simulink model "OFDM_USRP_Tx_Start"  (R2026a)
settings: Solver=FixedStepDiscrete  StopTime=inf  EnableMultiTasking=on
model workspace: external: MAT-File (data not in the file)
libraries: commdigbbndpm3 x2, dspxfrm3 x1, commfilt2 x1
settings Model: SimulationMode=accelerator  Creator=thua3267  LastModifiedBy=dawn

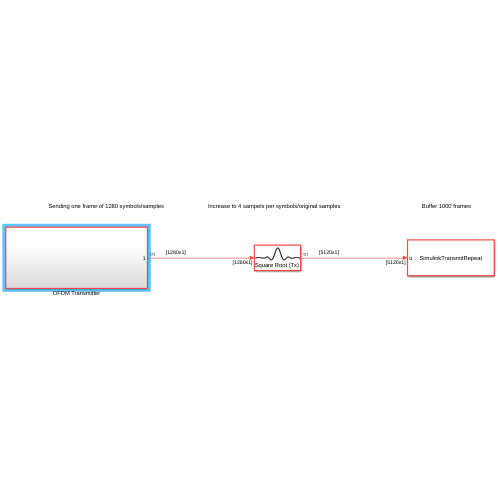
[thumbnail: Simulink's stored preview of the top-level diagram]
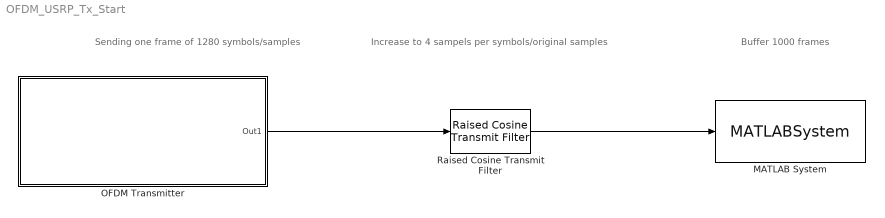
== system OFDM_USRP_Tx_Start ==
  note: Sending one frame of 1280 symbols/samples
  note: Increase to 4 sampels per symbols/original samples
  note: Buffer 1000 frames
  MATLAB System : MATLABSystem  System=SimulinkTransmitRepeat  Platform=X310  SerialNum=30AABDE  ChannelMapping=1  CenterFrequency=921e6  LocalOscillatorOffset=0  Gain=60  PPSSource=Internal  ClockSource=Internal  MasterClockRate=184.32e6  InterpolationFactor=72
      mask Type: SimulinkTransmitRepeat
  OFDM Transmitter : Subsystem
  Raised Cosine Transmit Filter : commfilt2/Raised Cosine Transmit Filter  filtType=Square root  R=0.5  filtSpan=10  N=4  filterGain=1  InputProcessing=Columns as channels (frame based)  RateOptions=Enforce single-rate processing  framing=Mute  checkCoeff=off  variableName=rcTxFilt1  checkGain=Normalized  sampMode=Mute  saveAsFlag=0  currentFiltSpan=10  D=(10)/2  launchFVT=off  roundingMode=Floor  overflowMode=off  coeffDataTypeStr=Inherit: Same word length as input  coeffMin=[]  coeffMax=[]  coeffLastDataTypeStr=Inherit: Same word length as input  outputDataTypeStr=Inherit: Same as accumulator  outputMin=[]  outputMax=[]  outputLastDataTypeStr=Inherit: Same as accumulator
  wires:
  OFDM Transmitter/1(Out1) -> Raised Cosine Transmit Filter/1
  Raised Cosine Transmit Filter/1 -> MATLAB System/1

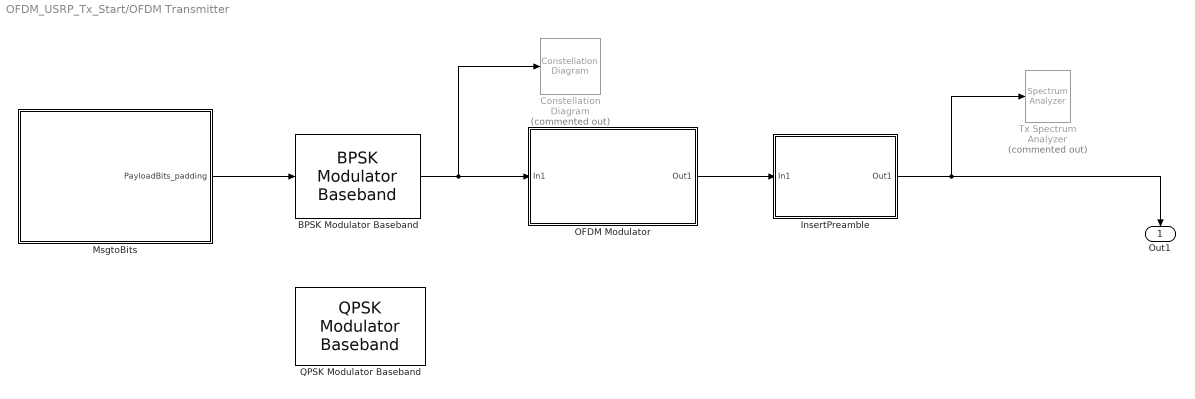
== system OFDM_USRP_Tx_Start/OFDM Transmitter ==
  BPSK Modulator Baseband : commdigbbndpm3/BPSK Modulator Baseband  Ph=0  outDtype=double  outWordLen=16  outUDDataType=sfix(16)  outFracLenMode=Best precision  outFracLen=15  outDataTypeStr=double  outLastDataTypeStr=double
  Constellation Diagram : ConstellationDiagram  Commented=on  WindowPosition=[1 41 1920 964]  DefaultConfigurationName=comm.scopes.ConstellationDiagramBlockCfg
  InsertPreamble : Subsystem
  MsgtoBits : MATLAB Function  TreatAsAtomicUnit=on
  OFDM Modulator : Subsystem
  QPSK Modulator Baseband : commdigbbndpm3/QPSK Modulator Baseband  InType=Integer  Enc=Gray  Ph=pi/4  outDtype=double  outWordLen=16  outUDDataType=sfix(16)  outFracLenMode=Best precision  outFracLen=15  outDataTypeStr=double  outLastDataTypeStr=double
  Tx Spectrum Analyzer : SpectrumAnalyzer  Commented=on  WindowPosition=[2288 304 800 592]  Method=Welch  SampleRate=6400  Span=6400  StartFrequency=-3200  StopFrequency=3200  AveragingMethod=Running  YLimits=[-75.98895818008306,-0.83072294749134024]  AllowFFTLengthLessThanSamplesPerUpdate=on  DefaultConfigurationName=spbscopes.SpectrumAnalyzerBlockCfg  IsFrequencyInputMode=0  FrequencyVectorPort=0  FrequencyVectorFromPort=0  FrequencyInputRBWPort=0  FrequencyInputRBWFromPort=0
  Out1 : Outport  VectorParamsAs1DForOutWhenUnconnected=off
  wires:
  MsgtoBits/1(PayloadBits_padding) -> BPSK Modulator Baseband/1
  InsertPreamble/1(Out1) -> Out1/1, Tx Spectrum Analyzer/1
  BPSK Modulator Baseband/1 -> Constellation Diagram/1, OFDM Modulator/1(In1)
  OFDM Modulator/1(Out1) -> InsertPreamble/1(In1)

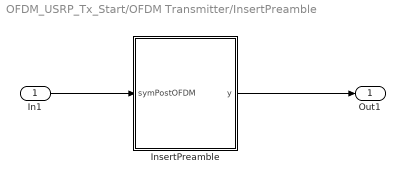
== system OFDM_USRP_Tx_Start/OFDM Transmitter/InsertPreamble ==
  In1 : Inport
  InsertPreamble : MATLAB Function  TreatAsAtomicUnit=on
  Out1 : Outport  VectorParamsAs1DForOutWhenUnconnected=off
  wires:
  InsertPreamble/1(y) -> Out1/1
  In1/1 -> InsertPreamble/1(symPostOFDM)

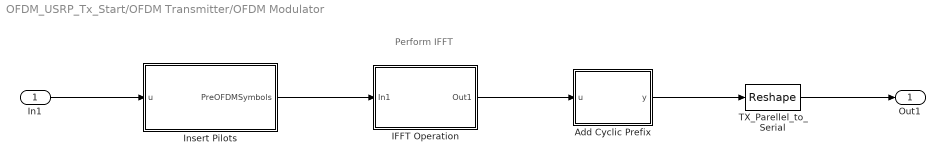
== system OFDM_USRP_Tx_Start/OFDM Transmitter/OFDM Modulator ==
  note: Perform IFFT
  In1 : Inport
  " TX_Parellel_to_Serial" : Reshape  OutputDimensionality=Column vector (2-D)
  Add Cyclic Prefix : MATLAB Function  TreatAsAtomicUnit=on
  IFFT Operation : Subsystem
  Insert Pilots : MATLAB Function  TreatAsAtomicUnit=on
  Out1 : Outport  VectorParamsAs1DForOutWhenUnconnected=off
  wires:
  " TX_Parellel_to_Serial"/1 -> Out1/1
  Add Cyclic Prefix/1(y) -> " TX_Parellel_to_Serial"/1
  In1/1 -> Insert Pilots/1(u)
  Insert Pilots/1(PreOFDMSymbols) -> IFFT Operation/1(In1)
  IFFT Operation/1(Out1) -> Add Cyclic Prefix/1(u)

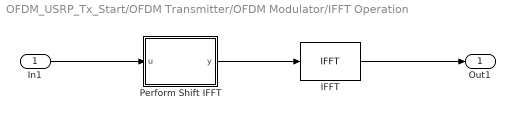
== system OFDM_USRP_Tx_Start/OFDM Transmitter/OFDM Modulator/IFFT Operation ==
  In1 : Inport
  IFFT : dspxfrm3/IFFT  FFTImplementation=Auto  CompMethod=Table lookup  TableOpt=NEW  TableOptActive=Speed  BitRevOrder=off  cs_in=off  Normalize=on  InheritFFTLength=on  FFTLength=64  WrapInput=on  mode=Complex  outSamplingMode=Sample based  roundingMode=Floor  overflowMode=off  firstCoeffDataTypeStr=Inherit: Same word length as input  firstCoeffLastDataTypeStr=Inherit: Same word length as input  outputMin=[]  outputMax=[]
  Perform Shift IFFT : MATLAB Function  TreatAsAtomicUnit=on
  Out1 : Outport  VectorParamsAs1DForOutWhenUnconnected=off
  wires:
  IFFT/1 -> Out1/1
  In1/1 -> Perform Shift IFFT/1(u)
  Perform Shift IFFT/1(y) -> IFFT/1

== matlab function OFDM_USRP_Tx_Start/OFDM Transmitter/OFDM Modulator/Insert Pilots ==
  data: u input; PreOFDMSymbols output
function PreOFDMSymbols = InsertPilots(u)
%INSERTPILOTS Map payload data and pilots onto the 64-point OFDM grid.
%
%   PreOFDMSymbols = InsertPilots(u)
%
%   INPUT
%       u              : 576x1 complex payload (48 data carriers x 12 OFDM symbols)
%
%   OUTPUT
%       PreOFDMSymbols : 64x12 frequency-domain grid, ready for the IFFT
%                        (pilots on 4 carriers, data on 48, rest = guard/DC = 0)

% System parameters
NumOFDMSymbols  = 12;
NumDataCarriers = 48;   % OFDM data carriers

% OFDM parameters
FFTlen = 64;
PilotCarrierIndices = [12;26;40;54];                          % length = 4
DataCarrierIndices  = [7:11,13:25,27:32,34:39,41:53,55:59]';  % length = 48, assuming DC at carrier 33
% GuardBandCarriers = [1:6, 60:64]';                          % length = 11

% Get pilots for each frame
coder.extrinsic('getOFDMPreambleAndPilot_mymodel');
Pilots = coder.const(double(getOFDMPreambleAndPilot_mymodel('Pilot', NumOFDMSymbols)));

% Reshape input payload data with padding
ReshapedPayload = reshape(u, NumDataCarriers, NumOFDMSymbols);

% PreOFDMSymbols allocation
PreOFDMSymbols = complex(zeros(FFTlen, NumOFDMSymbols));
PreOFDMSymbols(PilotCarrierIndices, :) = Pilots;
PreOFDMSymbols(DataCarrierIndices,  :) = ReshapedPayload;

end

== matlab function OFDM_USRP_Tx_Start/OFDM Transmitter/MsgtoBits ==
  data: PayloadBits_padding output
function PayloadBits_padding   = MsgtoBits
%This function converts a message to payloadBits with padding 

%% Configuration paramters
%System Paramters
   NumDataCarriers = 48;%OFDM data carriers
   NumBitsPerCharacter  = 7;
   BitsPerSymbol = 2; %bpsk 1, qpsk 2, 8qam 3;
   
%% Alogrithm 
%Payload message
    PayloadMessage = 'Welcome to the school of Electrical and Computer Engineering, Uni. of Sydney!';
    
%Convert message to bits
    coder.extrinsic('dec2bin');
    msgInBits = coder.const(double(dec2bin(PayloadMessage, NumBitsPerCharacter).'));
    PayloadBits = msgInBits(:) - 48;

% Calculate number of OFDM symbols per frame
   NumOFDMSymbols = 12; %ceil(length(PayloadBits)/BitsPerSymbol/NumDataCarriers);
   
% Calculate number of bits padded in each frame
   NumPadSymbols = NumDataCarriers * NumOFDMSymbols - length(PayloadBits)/BitsPerSymbol; %# of padded symbols required
   NumPadBits = NumPadSymbols * BitsPerSymbol; %# of padded bits required
    
%  PayloadBits with padding
    PayloadBits_padding = [PayloadBits; zeros(NumPadBits, 1)];

== matlab function OFDM_USRP_Tx_Start/OFDM Transmitter/InsertPreamble/InsertPreamble ==
  data: y output size=[1280,1]; symPostOFDM input
function y = InsertPreamble(symPostOFDM)
%% Configuration paramters
FFTLength=64;
NumGuardBandCarriers = [6; 5];
NumFrames=1;

%% Alorithm
%Get preamble for each frame
coder.extrinsic('getOFDMPreambleAndPilot_mymodel');
Preamble = coder.const(double(getOFDMPreambleAndPilot_mymodel('Preamble', FFTLength, NumGuardBandCarriers)));

% Repeat the frame
 y = repmat([Preamble; symPostOFDM], NumFrames, 1);%in general set NumFrames = 1. Let Block Buffer to repeat # of frames

== matlab function OFDM_USRP_Tx_Start/OFDM Transmitter/OFDM Modulator/Add Cyclic Prefix ==
  data: u input; y output
function y = addCycPrefix(u)
%ADDCYCPREFIX Add a cyclic prefix of length 16 to each OFDM symbol (Add Cyclic Prefix block).
%
%   y = addCycPrefix(u)
%
%   INPUT
%       u : 64x12 complex matrix, IFFT output (FFTlen x NumOFDMSymbols).
%           Each column is one OFDM symbol.
%
%   OUTPUT
%       y : 80x12 complex matrix, each column = [last 16 samples of u(:,k); u(:,k)]
%           (768 samples -> 960 samples). The next block, Parallel to Series,
%           converts this 80x12 matrix to a 960x1 vector.

% Configuration parameters
FFTlen         = 64;
NumOFDMSymbols = 12;
CPlen          = 16;

% Algorithm
u = reshape(u, FFTlen, NumOFDMSymbols);

% Copy the last CPlen samples of every symbol (column) ...
CP = u(FFTlen-CPlen+1:FFTlen, :);     % 16 x 12

% ... and prepend them to the symbol
y = [CP; u];                           % 80 x 12

end

== matlab function OFDM_USRP_Tx_Start/OFDM Transmitter/OFDM Modulator/IFFT Operation/Perform Shift IFFT ==
  data: u input; y output
function y = shiftIFFT(u)
y=ifftshift(u,1);
